simulink model "Project1"  (R2025b)
settings: Solver=VariableStepAuto  StartTime=0.0  StopTime=10.0  RelTol=1e-3
settings Model: Creator=hendl  LastModifiedBy=hendl

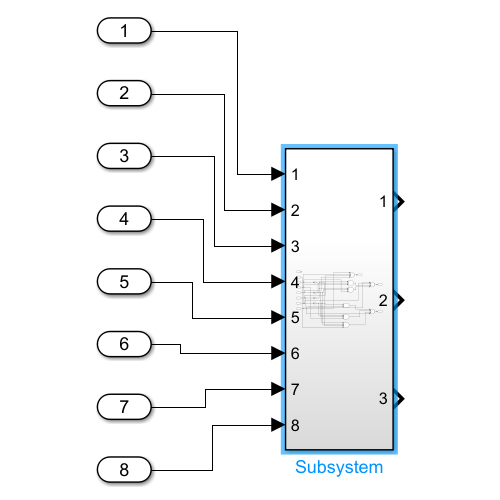
[thumbnail: Simulink's stored preview of the top-level diagram]
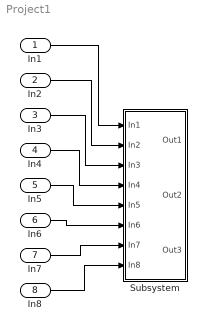
== system Project1 ==
  In1 : Inport
  In2 : Inport  Port=2
  In3 : Inport  Port=3
  In4 : Inport  Port=4
  In5 : Inport  Port=5
  In6 : Inport  Port=6
  In7 : Inport  Port=7
  In8 : Inport  Port=8
  Subsystem : Subsystem
  wires:
  In1/1 -> Subsystem/1(In1)
  In2/1 -> Subsystem/2(In2)
  In3/1 -> Subsystem/3(In3)
  In4/1 -> Subsystem/4(In4)
  In5/1 -> Subsystem/5(In5)
  In6/1 -> Subsystem/6(In6)
  In7/1 -> Subsystem/7(In7)
  In8/1 -> Subsystem/8(In8)

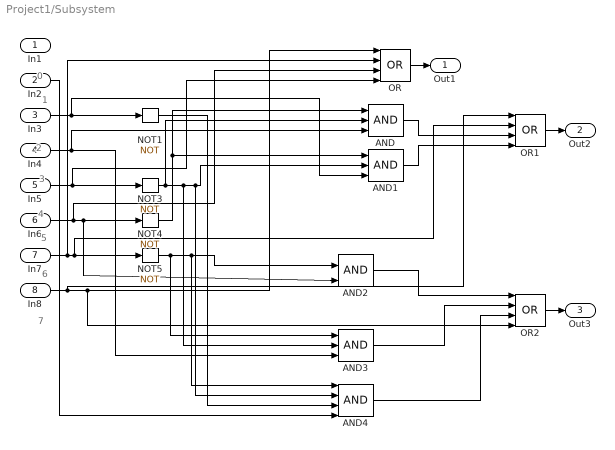
== system Project1/Subsystem ==
  note: 7
  note: 6
  note: 5
  note: 4
  note: 3
  note: 2
  note: 1
  note: 0
  In1 : Inport
  In2 : Inport  Port=2
  In3 : Inport  Port=3
  In4 : Inport  Port=4
  In5 : Inport  Port=5
  In6 : Inport  Port=6
  In7 : Inport  Port=7
  In8 : Inport  Port=8
  AND : Logic  Inputs=3  IconShape=distinctive  AllPortsSameDT=off  OutDataTypeStr=boolean
  AND1 : Logic  Inputs=3  IconShape=distinctive  AllPortsSameDT=off  OutDataTypeStr=boolean
  AND2 : Logic  IconShape=distinctive  AllPortsSameDT=off  OutDataTypeStr=boolean
  AND3 : Logic  Inputs=3  IconShape=distinctive  AllPortsSameDT=off  OutDataTypeStr=boolean
  AND4 : Logic  Inputs=4  IconShape=distinctive  AllPortsSameDT=off  OutDataTypeStr=boolean
  NOT{1,3..5} (4 alike) : Logic  Operator=NOT  IconShape=distinctive  AllPortsSameDT=off  OutDataTypeStr=boolean
  OR : Logic  Operator=OR  Inputs=4  IconShape=distinctive  AllPortsSameDT=off  OutDataTypeStr=boolean
  OR1 : Logic  Operator=OR  Inputs=4  IconShape=distinctive  AllPortsSameDT=off  OutDataTypeStr=boolean
  OR2 : Logic  Operator=OR  Inputs=4  IconShape=distinctive  AllPortsSameDT=off  OutDataTypeStr=boolean
  Out1 : Outport
  Out2 : Outport  Port=2
  Out3 : Outport  Port=3
  wires:
  AND4/1 -> OR2/3
  NOT5/1 -> AND3/1, AND4/1, AND2/1
  In7/1 -> OR/2, OR1/2, NOT5/1
  In8/1 -> OR1/1, OR2/4, OR/1
  AND/1 -> OR1/3
  In2/1 -> AND4/4
  OR/1 -> Out1/1
  In5/1 -> OR/4, NOT3/1
  NOT4/1 -> AND1/1, AND/1
  NOT1/1 -> AND4/3
  OR2/1 -> Out3/1
  In4/1 -> AND/3, AND3/3
  AND3/1 -> OR2/2
  NOT3/1 -> AND3/2, AND4/2, AND1/2, AND/2
  In6/1 -> OR/3, AND2/2, NOT4/1
  In3/1 -> AND1/3, NOT1/1
  AND1/1 -> OR1/4
  AND2/1 -> OR2/1
  OR1/1 -> Out2/1
